simulink model "bldc_model"  (R2025b)
settings: Solver=FixedStepDiscrete  StartTime=0.0  StopTime=50  FixedStep=0.01  MaxStep=1e-4  RelTol=1e-3  EnableMultiTasking=on
libraries: simulink x2, c29H85xlib x1
settings Model: ExtModeTrigDuration=2  Creator=FOFIEVIGOLBRYAN  LastModifiedBy=FOFIEVIGOLBRYAN
settings SolverCC: AutoInsertRateTranBlk=on
settings OptimizationCC: EnhancedBackFolding=on  PassReuseOutputArgsAs=Individual arguments  ZeroExternalMemoryAtStartup=off  ZeroInternalMemoryAtStartup=off  MaxStackSize=64  OptimizeBlockOrder=speed  DifferentSizesBufferReuse=on  OptimizationCustomize=off  EfficientTunableParamExpr=on
settings DebuggingCC: ParameterTunabilityLossMsg=error
settings HardwareCC: ProdBitPerPointer=32.0  ProdBitPerSizeT=32.0  ProdBitPerPtrDiffT=32.0  ProdLargestAtomicInteger=Long  ProdLargestAtomicFloat=Double  ProdWordSize=32.0  ProdHWDeviceType=ARM Compatible->ARM Cortex
settings SFSimCC: MATLABDynamicMemAlloc=off
settings RTWCC: SystemTargetFile=ert.tlc  HardwareBoard=ESP32-WROOM (Arduino Compatible)  TLCOptions="-aInlineSetEventsForThisBaseRateFcn=TLC_FALSE -aSuppressMultiTaskScheduler=TLC_FALSE  -aRateBasedStepFcn=0"  TemplateMakefile=ert_default_tmf  Toolchain=ESP32  BuildConfiguration=Faster Runs  Description=Embedded Coder
settings CodeAppCC: ForceParamTrailComments=on  IgnoreCustomStorageClasses=off  OperatorAnnotations=on  SimulinkDataObjDesc=on  SFDataObjDesc=on  InsertBlockDesc=on
settings ERTTargetCC: ExtModeTransport=3.0  ExtModeStaticAlloc=on  ExtModeAutomaticAllocSize=off  ExtModeStaticAllocSize=65536.0  ExtModeMexFile=ext_xcp  ExtModeIntrfLevel=Level2 - Open  InlinedParameterPlacement=Hierarchical  SupportContinuousTime=on  SupportVariableSizeSignals=on

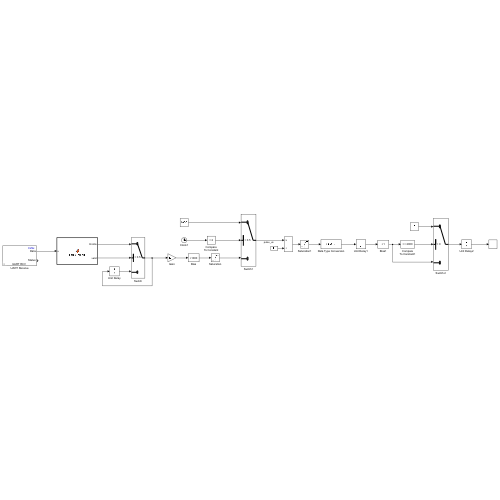
[thumbnail: Simulink's stored preview of the top-level diagram]
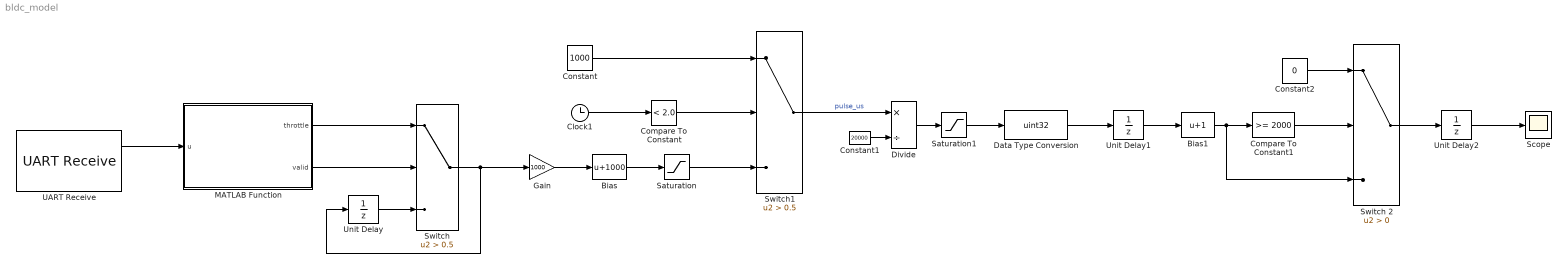
== system bldc_model ==
  Bias : Bias  Bias=1000  SaturateOnIntegerOverflow=off
  Bias1 : Bias  Bias=1  SaturateOnIntegerOverflow=off
  Clock1 : Clock
  Compare To Constant : simulink/Logic and Bit Operations/Compare To Constant  relop=<  const=2.0  OutDataTypeStr=boolean
  Compare To Constant1 : simulink/Logic and Bit Operations/Compare To Constant  relop=>=  const=2000  OutDataTypeStr=boolean
  Constant : Constant  Value=1000
  Constant1 : Constant  Value=20000
  Constant2 : Constant  Value=0
  Data Type Conversion : DataTypeConversion  OutDataTypeStr=uint32  SaturateOnIntegerOverflow=off  RndMeth=Floor
  Divide : Product  Inputs=*/
  Gain : Gain  Gain=1000
  MATLAB Function : MATLAB Function  TreatAsAtomicUnit=on
  Saturation : Saturate  UpperLimit=2000  LowerLimit=1000
  Saturation1 : Saturate  UpperLimit=0.10  LowerLimit=0.05
  Scope : Scope
  Switch : Switch  Criteria=u2 > Threshold  Threshold=0.5  SaturateOnIntegerOverflow=off  InputSameDT=off
  Switch 2 : Switch  Criteria=u2 > Threshold  SaturateOnIntegerOverflow=off  InputSameDT=off
  Switch1 : Switch  Criteria=u2 > Threshold  Threshold=0.5  SaturateOnIntegerOverflow=off  InputSameDT=off
  UART Receive : c29H85xlib/UART Receive  UartModule=A  UartPort=UART0  DataType=uint8  DataLength=32  SampleTime=0.01  OscillatorFreq=100  BlockingMode=off  BaudRate=115207.3733  StopBits=0  ParityMode=NONE  PinAssignment_Rx=85
  Unit Delay : UnitDelay  SampleTime=-1  HasFrameUpgradeWarning=on
  Unit Delay1 : UnitDelay  SampleTime=1e-5  HasFrameUpgradeWarning=on
  Unit Delay2 : UnitDelay  SampleTime=1e-5  HasFrameUpgradeWarning=on
  wires:
  MATLAB Function/1(throttle) -> Switch/1
  MATLAB Function/2(valid) -> Switch/2
  Clock1/1 -> Compare To Constant/1
  Compare To Constant/1 -> Switch1/2
  Switch/1 -> Unit Delay/1, Gain/1
  Unit Delay/1 -> Switch/3
  Constant/1 -> Switch1/1
  Bias/1 -> Saturation/1
  Gain/1 -> Bias/1
  Saturation/1 -> Switch1/3
  UART Receive/1 -> MATLAB Function/1(u)
  Switch1/1 -> Divide/1  "pulse_us"
  Constant1/1 -> Divide/2
  Divide/1 -> Saturation1/1
  Saturation1/1 -> Data Type Conversion/1
  Unit Delay1/1 -> Bias1/1
  Bias1/1 -> Switch 2/3, Compare To Constant1/1
  Compare To Constant1/1 -> Switch 2/2
  Constant2/1 -> Switch 2/1
  Data Type Conversion/1 -> Unit Delay1/1
  Switch 2/1 -> Unit Delay2/1
  Unit Delay2/1 -> Scope/1

== matlab function bldc_model/MATLAB Function ==
  data: u input; throttle output; valid output
function [throttle, valid] = parseThrottle(u)
% u: uint8 buffer (ASCII). Expected: 'T,0.35\n'
% throttle: single 0..1
% valid: true if message parsed correctly

valid = false;
throttle = single(0);

% Convert to char, remove zeros
c = char(u(:))';
c(c==0) = [];

% Find 'T,' pattern
idx = strfind(c, 'T,');
if isempty(idx)
    return;
end

% Extract after 'T,' until newline
start = idx(end) + 2;
nl = find(c(start:end) == newline, 1, 'first');
cr = find(c(start:end) == char(13), 1, 'first'); % \r

stop = [];
if ~isempty(nl), stop = start + nl - 2; end
if isempty(stop) && ~isempty(cr), stop = start + cr - 2; end
if isempty(stop)
    % No terminator found, try to parse until end
    stop = length(c);
end

numstr = strtrim(c(start:stop));
v = str2double(numstr);

if ~isnan(v)
    % saturate 0..1
    if v < 0, v = 0; end
    if v > 1, v = 1; end
    throttle = single(v);
    valid = true;
end
end
